simulink model "FAST_11TO14mpers"  (R2019a)
settings: Solver=FixedStepAuto  StartTime=0.0  StopTime=400  FixedStep=DT  RelTol=1e-3
values from neighbouring files (symbols this model uses):
  Control = struct    [testqLPV.m]
  Drivetrain = struct    [dataDLR.m]
  OutList = OutTable.Properties.VariableNames    [initLPVParam.m]    (also in testCtrl.m; testOutList.m = cell(40, 1); testqLPV.m = cell(40, 1))
undefined symbols (not defined in the file or in its folder): CertificationSettings, DiscIntNeverNeededParam, P_InitAngle, RPM_Init, strmatch
settings Model: ExtModeTrigMode=oneshot  ExtModeArmWhenConnect=off  Creator=Hazim Namik  LastModifiedBy=ditt_aj
settings DataIOCC: LimitDataPoints=on  SaveFormat=Array  ReturnWorkspaceOutputs=off
settings OptimizationCC: BlockReduction=off  BooleanDataType=off  LifeSpan=inf
settings DebuggingCC: SaveWithParameterizedLinksMsg=none  UnderspecifiedInitializationDetection=Classic  MergeDetectMultiDrivingBlocksExec=none  SignalResolutionControl=TryResolveAllWithWarning  SFUnexpectedBacktrackingDiag=warning  SFNoUnconditionalDefaultTransitionDiag=warning  SFExecutionAtInitializationDiag=none  ArithmeticOperatorsInVariantConditions=warning
settings HardwareCC: ProdBitPerPointer=32  ProdBitPerSizeT=32  ProdBitPerPtrDiffT=32  ProdLargestAtomicFloat=None  ProdIntDivRoundTo=Undefined  ProdEndianess=Unspecified  ProdWordSize=32  ProdHWDeviceType=32-bit Generic  TargetUnknown=on
settings ModelReferenceCC: PropagateSignalLabelsOutOfModel=off
settings SFSimCC: SimUseLocalCustomCode=off
settings RTWCC: RTWUseLocalCustomCode=off
settings CodeAppCC: StateflowObjectComments=on
settings GRTTargetCC: TargetLangStandard=C89/C90 (ANSI)  GeneratePreprocessorConditionals=Disable all
settings ConfigComp: CovMetricSettings=dw  CovHtmlReporting=on  CovSaveCumulativeToWorkspaceVar=on  CovSaveSingleToWorkspaceVar=on  CovExternalEMLEnable=off

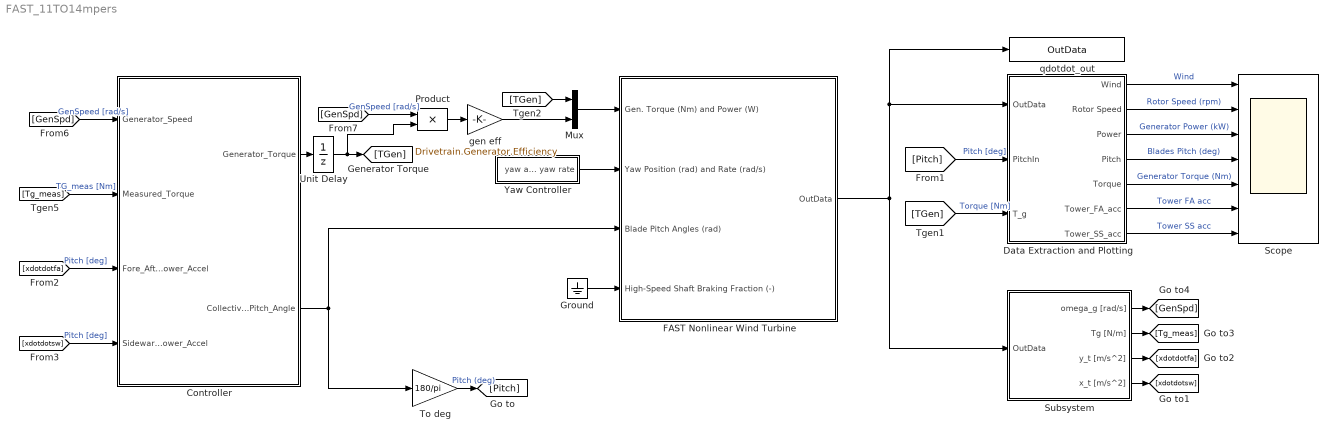
== system FAST_11TO14mpers ==
  Controller : Subsystem
  Data Extraction and Plotting : Subsystem
  FAST Nonlinear Wind Turbine : Subsystem  mask(FAST Nonlinear Wind Turbine){}
      mask help: This block contains the FAST S-Function.
      mask init:
      | clear FAST_SFunc
  Ground : Ground
  Mux : Mux  Inputs=2
  Product : Product  RndMeth=Zero
  Scope : Scope  NumInputPorts=7
      settings: Tag=Scope
  Subsystem : Subsystem
  To deg : Gain  Gain=180/pi
  Unit Delay : UnitDelay  InitialCondition=RPM_Init*Drivetrain.Gearbox.Ratio  SampleTime=-1  HasFrameUpgradeWarning=on
  Yaw Controller : Subsystem
  gen eff : Gain  Gain=Drivetrain.Generator.Efficiency
  qdotdot_out : ToWorkspace  VariableName=OutData  SampleTime=-1
  wires:
  Mux/1 -> FAST Nonlinear Wind Turbine/1(Gen. Torque (Nm) and Power (W))
  Yaw Controller/1(yaw and yaw rate) -> FAST Nonlinear Wind Turbine/2(Yaw Position (rad) and Rate (rad/s))
  To deg/1 -> [Pitch]  "Pitch (deg)"
  gen eff/1 -> Mux/2
  Product/1 -> gen eff/1
  Data Extraction and Plotting/3(Power) -> Scope/3  "Generator Power (kW)"
  [Pitch] -> Data Extraction and Plotting/2(PitchIn)  "Pitch [deg]"
  Data Extraction and Plotting/1(Wind) -> Scope/1  "Wind"
  Data Extraction and Plotting/2(Rotor Speed) -> Scope/2  "Rotor Speed (rpm)"
  [TGen] -> Data Extraction and Plotting/3(T_g)  "Torque [Nm]"
  FAST Nonlinear Wind Turbine/1(OutData) -> qdotdot_out/1, Data Extraction and Plotting/1(OutData), Subsystem/1(OutData)
  Data Extraction and Plotting/4(Pitch) -> Scope/4  "Blades Pitch (deg)"
  Data Extraction and Plotting/5(Torque) -> Scope/5  "Generator Torque (Nm)"
  Controller/1(Generator_Torque) -> Unit Delay/1
  Controller/2(Collective_Pitch_Angle) -> FAST Nonlinear Wind Turbine/3(Blade Pitch Angles (rad)), To deg/1
  Data Extraction and Plotting/6(Tower_FA_acc) -> Scope/6  "Tower FA acc"
  Data Extraction and Plotting/7(Tower_SS_acc) -> Scope/7  "Tower SS acc"
  Ground/1 -> FAST Nonlinear Wind Turbine/4(High-Speed Shaft Braking Fraction (-))
  [TGen] -> Mux/1
  Unit Delay/1 -> Product/2, [TGen]
  Subsystem/1(omega_g [rad/s]) -> [GenSpd]
  Subsystem/3(y_t [m/s^2]) -> [xdotdotfa]
  Subsystem/4(x_t [m/s^2]) -> [xdotdotsw]
  [GenSpd] -> Controller/1(Generator_Speed)  "GenSpeed [rad/s]"
  [Tg_meas] -> Controller/2(Measured_Torque)  "TG_meas [Nm]"
  [xdotdotsw] -> Controller/4(Sidewards_Tower_Accel)  "Pitch [deg]"
  [xdotdotfa] -> Controller/3(Fore_Aft_Tower_Accel)  "Pitch [deg]"
  Subsystem/2(Tg [N/m]) -> [Tg_meas]
  [GenSpd] -> Product/1  "GenSpeed [rad/s]"

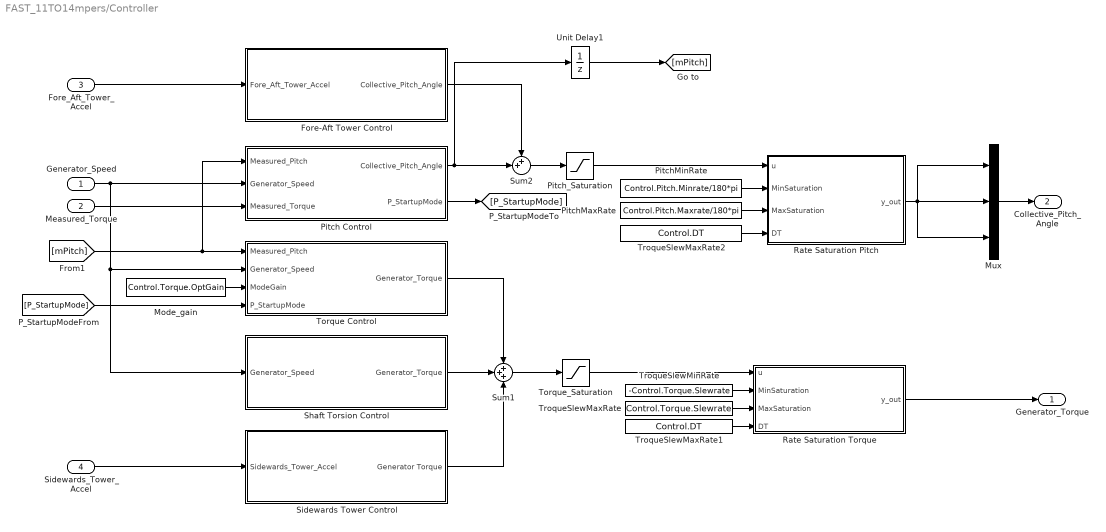
== system FAST_11TO14mpers/Controller ==
  Generator_Speed : Inport
  Measured_Torque : Inport  Port=2
  Fore_Aft_Tower_Accel : Inport  Port=3
  Sidewards_Tower_Accel : Inport  Port=4  PortDimensions=1
  Fore-Aft Tower Control : Subsystem
  Mode_gain : Constant  Value=Control.Torque.OptGain
  Mux : Mux  Inputs=3
  Pitch Control : Subsystem
  PitchMaxRate : Constant  Value=Control.Pitch.Maxrate/180*pi
  PitchMinRate : Constant  Value=Control.Pitch.Minrate/180*pi
  Pitch_Saturation : Saturate  UpperLimit=Control.Pitch.Max*pi/180  LowerLimit=Control.Pitch.Min*pi/180
  Rate Saturation Pitch : MATLAB Function  TreatAsAtomicUnit=on
  Rate Saturation Torque : MATLAB Function  TreatAsAtomicUnit=on
  Shaft Torsion Control : Subsystem
  Sidewards Tower Control : Subsystem
  Sum1 : Sum  Inputs=+++
  Sum2 : Sum  Inputs=++|
  Torque Control : Subsystem
  Torque_Saturation : Saturate  UpperLimit=Control.Torque.Limit  LowerLimit=Control.Torque.Min
  TroqueSlewMaxRate : Constant  Value=Control.Torque.Slewrate
  TroqueSlewMaxRate1 : Constant  Value=Control.DT
  TroqueSlewMaxRate2 : Constant  Value=Control.DT
  TroqueSlewMinRate : Constant  Value=-Control.Torque.Slewrate
  Unit Delay1 : UnitDelay  InitialCondition=P_InitAngle*pi/180  SampleTime=-1  HasFrameUpgradeWarning=on
  Generator_Torque : Outport
  Collective_Pitch_Angle : Outport  Port=2  PortDimensions=3
  wires:
  Sidewards_Tower_Accel/1 -> Sidewards Tower Control/1(Sidewards_Tower_Accel)
  Fore_Aft_Tower_Accel/1 -> Fore-Aft Tower Control/1(Fore_Aft_Tower_Accel)
  Fore-Aft Tower Control/1(Collective_Pitch_Angle) -> Sum2/1
  Torque Control/1(Generator_Torque) -> Sum1/1
  Sidewards Tower Control/1(Generator Torque) -> Sum1/3
  [mPitch] -> Pitch Control/1(Measured_Pitch), Torque Control/1(Measured_Pitch)
  Measured_Torque/1 -> Pitch Control/3(Measured_Torque)
  Shaft Torsion Control/1(Generator_Torque) -> Sum1/2
  Mode_gain/1 -> Torque Control/3(ModeGain)
  Sum1/1 -> Torque_Saturation/1
  Mux/1 -> Collective_Pitch_Angle/1
  Unit Delay1/1 -> [mPitch]
  Sum2/1 -> Pitch_Saturation/1
  Rate Saturation Pitch/1(y_out) -> Mux/3, Mux/2, Mux/1
  PitchMinRate/1 -> Rate Saturation Pitch/2(MinSaturation)
  PitchMaxRate/1 -> Rate Saturation Pitch/3(MaxSaturation)
  Pitch_Saturation/1 -> Rate Saturation Pitch/1(u)
  Torque_Saturation/1 -> Rate Saturation Torque/1(u)
  TroqueSlewMinRate/1 -> Rate Saturation Torque/2(MinSaturation)
  TroqueSlewMaxRate/1 -> Rate Saturation Torque/3(MaxSaturation)
  Generator_Speed/1 -> Pitch Control/2(Generator_Speed), Torque Control/2(Generator_Speed), Shaft Torsion Control/1(Generator_Speed)
  [P_StartupMode] -> Torque Control/4(P_StartupMode)
  Pitch Control/2(P_StartupMode) -> [P_StartupMode]
  Pitch Control/1(Collective_Pitch_Angle) -> Sum2/2, Unit Delay1/1
  Rate Saturation Torque/1(y_out) -> Generator_Torque/1
  TroqueSlewMaxRate1/1 -> Rate Saturation Torque/4(DT)
  TroqueSlewMaxRate2/1 -> Rate Saturation Pitch/4(DT)

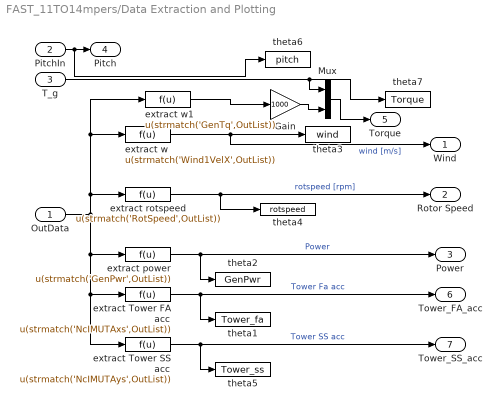
== system FAST_11TO14mpers/Data Extraction and Plotting ==
  OutData : Inport
  PitchIn : Inport  Port=2
  T_g : Inport  Port=3
  Gain : Gain  Gain=1000
  Mux : Mux  Inputs=2
  extract Tower FA acc : Fcn  Expr=u(strmatch('NcIMUTAxs',OutList))
  extract Tower SS acc : Fcn  Expr=u(strmatch('NcIMUTAys',OutList))
  extract power : Fcn  Expr=u(strmatch('GenPwr',OutList))
  extract rotspeed : Fcn  Expr=u(strmatch('RotSpeed',OutList))
  extract w : Fcn  Expr=u(strmatch('Wind1VelX',OutList))
  extract w1 : Fcn  Expr=u(strmatch('GenTq',OutList))
  theta1 : ToWorkspace  VariableName=Tower_fa  SampleTime=-1
      settings: MaxDataPoints=Inf  Decimation=3
  theta2 : ToWorkspace  VariableName=GenPwr  SampleTime=-1
      settings: MaxDataPoints=Inf  Decimation=3
  theta3 : ToWorkspace  VariableName=wind  SampleTime=-1
      settings: MaxDataPoints=Inf  Decimation=3
  theta4 : ToWorkspace  VariableName=rotspeed  SampleTime=-1
      settings: MaxDataPoints=Inf  Decimation=3
  theta5 : ToWorkspace  VariableName=Tower_ss  SampleTime=-1
      settings: MaxDataPoints=Inf  Decimation=3
  theta6 : ToWorkspace  VariableName=pitch  SampleTime=-1
      settings: MaxDataPoints=Inf  Decimation=3
  theta7 : ToWorkspace  VariableName=Torque  SampleTime=-1
      settings: MaxDataPoints=Inf  Decimation=3
  Wind : Outport
  Rotor Speed : Outport  Port=2
  Power : Outport  Port=3
  Pitch : Outport  Port=4
  Torque : Outport  Port=5
  Tower_FA_acc : Outport  Port=6
  Tower_SS_acc : Outport  Port=7
  wires:
  extract w/1 -> Wind/1, theta3/1  "wind [m/s]"
  extract rotspeed/1 -> theta4/1, Rotor Speed/1  "rotspeed [rpm]"
  extract power/1 -> theta2/1, Power/1  "Power"
  PitchIn/1 -> theta6/1, Pitch/1
  T_g/1 -> Mux/1, theta7/1
  extract Tower FA acc/1 -> theta1/1, Tower_FA_acc/1  "Tower Fa acc"
  OutData/1 -> extract w/1, extract w1/1, extract rotspeed/1, extract Tower SS acc/1, extract Tower FA acc/1, extract power/1
  extract Tower SS acc/1 -> theta5/1, Tower_SS_acc/1  "Tower SS acc"
  extract w1/1 -> Gain/1
  Gain/1 -> Mux/2
  Mux/1 -> Torque/1

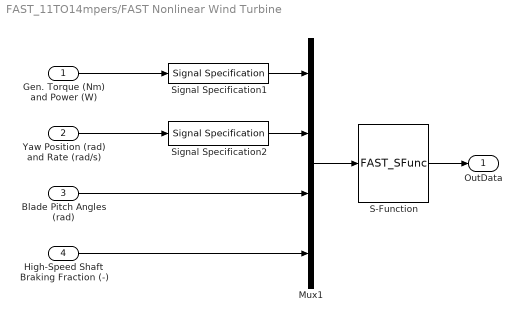
== system FAST_11TO14mpers/FAST Nonlinear Wind Turbine ==
  Gen. Torque (Nm) and Power (W) : Inport
  Yaw Position (rad) and Rate (rad/s) : Inport  Port=2
  Blade Pitch Angles (rad) : Inport  Port=3
  High-Speed Shaft Braking Fraction (-) : Inport  Port=4
  Mux1 : Mux
  S-Function : S-Function  FunctionName=FAST_SFunc  Parameters=FAST_InputFileName, TMax, 0  SFunctionDeploymentMode=off  EnableBusSupport=off
  Signal Specification1 : SignalSpecification  OutDataTypeStr=double  Dimensions=2
  Signal Specification2 : SignalSpecification  OutDataTypeStr=double  Dimensions=2
  OutData : Outport
  wires:
  Gen. Torque (Nm) and Power (W)/1 -> Signal Specification1/1
  S-Function/1 -> OutData/1
  Mux1/1 -> S-Function/1
  Blade Pitch Angles (rad)/1 -> Mux1/3
  Yaw Position (rad) and Rate (rad/s)/1 -> Signal Specification2/1
  Signal Specification1/1 -> Mux1/1
  Signal Specification2/1 -> Mux1/2
  High-Speed Shaft Braking Fraction (-)/1 -> Mux1/4

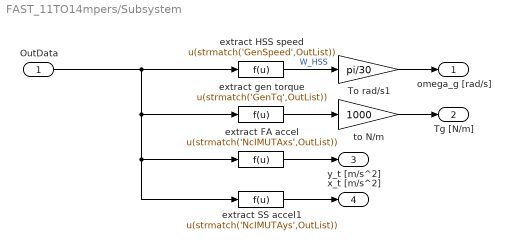
== system FAST_11TO14mpers/Subsystem ==
  OutData : Inport
  To rad/s1 : Gain  Gain=pi/30
  extract FA accel : Fcn  Expr=u(strmatch('NcIMUTAxs',OutList))
  extract HSS speed : Fcn  Expr=u(strmatch('GenSpeed',OutList))
  extract SS accel1 : Fcn  Expr=u(strmatch('NcIMUTAys',OutList))
  extract gen torque : Fcn  Expr=u(strmatch('GenTq',OutList))
  to N/m : Gain  Gain=1000
  omega_g [rad/s] : Outport
  Tg [N/m] : Outport  Port=2
  y_t [m/s^2] : Outport  Port=3
  x_t [m/s^2] : Outport  Port=4
  wires:
  to N/m/1 -> Tg [N/m]/1
  OutData/1 -> extract SS accel1/1, extract FA accel/1, extract gen torque/1, extract HSS speed/1
  extract FA accel/1 -> y_t [m/s^2]/1
  extract HSS speed/1 -> To rad/s1/1  "W_HSS"
  extract gen torque/1 -> to N/m/1
  extract SS accel1/1 -> x_t [m/s^2]/1
  To rad/s1/1 -> omega_g [rad/s]/1

== system FAST_11TO14mpers/Yaw Controller ==
  Mux : Mux  Inputs=2
  Yaw Position : Constant  Value=0
  Yaw rate : Constant  Value=0
  yaw and yaw rate : Outport
  wires:
  Mux/1 -> yaw and yaw rate/1
  Yaw Position/1 -> Mux/1
  Yaw rate/1 -> Mux/2

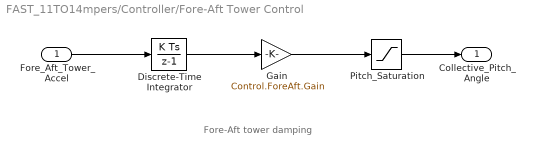
== system FAST_11TO14mpers/Controller/Fore-Aft Tower Control ==
  note: Fore-Aft tower damping
  Fore_Aft_Tower_Accel : Inport
  Discrete-Time Integrator : DiscreteIntegrator  SampleTime=-1  ICPrevOutput=DiscIntNeverNeededParam  ICPrevScaledInput=DiscIntNeverNeededParam
  Gain : Gain  Gain=Control.ForeAft.Gain
  Pitch_Saturation : Saturate  UpperLimit=Control.ForeAft.MaxPitchAmplitude*pi/180  LowerLimit=-Control.ForeAft.MaxPitchAmplitude*pi/180
  Collective_Pitch_Angle : Outport
  wires:
  Fore_Aft_Tower_Accel/1 -> Discrete-Time Integrator/1
  Pitch_Saturation/1 -> Collective_Pitch_Angle/1
  Discrete-Time Integrator/1 -> Gain/1
  Gain/1 -> Pitch_Saturation/1

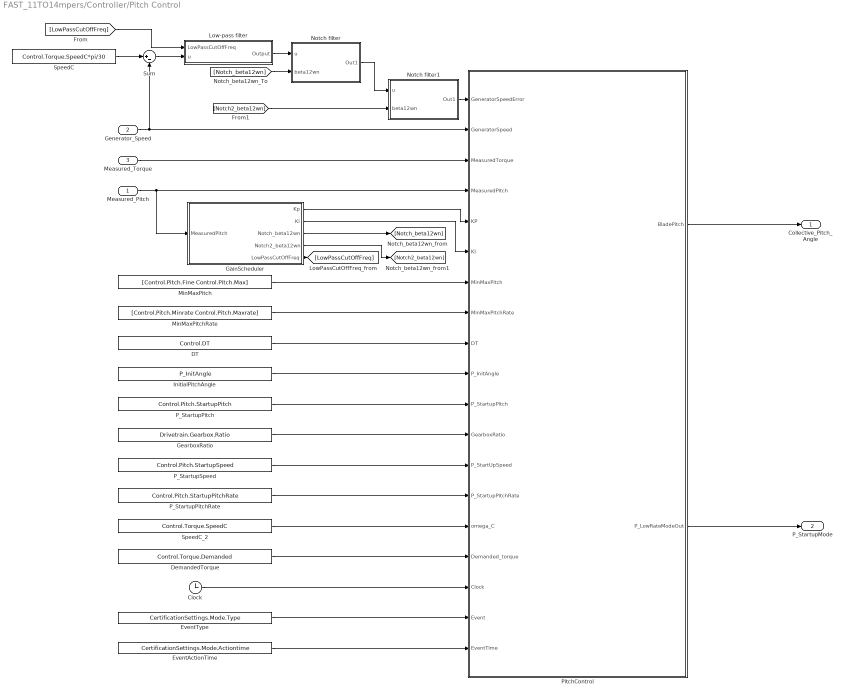
== system FAST_11TO14mpers/Controller/Pitch Control ==
  Measured_Pitch : Inport
  Generator_Speed : Inport  Port=2
  Measured_Torque : Inport  Port=3
  Clock : Clock
  DT : Constant  Value=Control.DT
  DemandedTorque : Constant  Value=Control.Torque.Demanded
  EventActionTime : Constant  Value=CertificationSettings.Mode.Actiontime
  EventType : Constant  Value=CertificationSettings.Mode.Type
  GainScheduler : Subsystem
  GearboxRatio : Constant  Value=Drivetrain.Gearbox.Ratio
  InitialPitchAngle : Constant  Value=P_InitAngle
  Low-pass filter : Subsystem
  MinMaxPitch : Constant  Value=[Control.Pitch.Fine Control.Pitch.Max]
  MinMaxPitchRate : Constant  Value=[Control.Pitch.Minrate Control.Pitch.Maxrate]
  Notch filter : Subsystem
  Notch filter1 : Subsystem
  P_StartupPitch : Constant  Value=Control.Pitch.StartupPitch
  P_StartupPitchRate : Constant  Value=Control.Pitch.StartupPitchRate
  P_StartupSpeed : Constant  Value=Control.Pitch.StartupSpeed
  PitchControl : MATLAB Function  TreatAsAtomicUnit=on
  SpeedC : Constant  Value=Control.Torque.SpeedC*pi/30
  SpeedC_2 : Constant  Value=Control.Torque.SpeedC
  Sum : Sum  Inputs=|+-
  Collective_Pitch_Angle : Outport
  P_StartupMode : Outport  Port=2
  wires:
  MinMaxPitch/1 -> PitchControl/7(MinMaxPitch)
  MinMaxPitchRate/1 -> PitchControl/8(MinMaxPitchRate)
  PitchControl/1(BladePitch) -> Collective_Pitch_Angle/1
  Measured_Torque/1 -> PitchControl/3(MeasuredTorque)
  SpeedC/1 -> Sum/1
  Generator_Speed/1 -> PitchControl/2(GeneratorSpeed), Sum/2
  Sum/1 -> Low-pass filter/2(u)
  PitchControl/2(P_LowRateModeOut) -> P_StartupMode/1
  DT/1 -> PitchControl/9(DT)
  P_StartupPitch/1 -> PitchControl/11(P_StartupPitch)
  InitialPitchAngle/1 -> PitchControl/10(P_InitAngle)
  GearboxRatio/1 -> PitchControl/12(GearboxRatio)
  P_StartupSpeed/1 -> PitchControl/13(P_StartUpSpeed)
  P_StartupPitchRate/1 -> PitchControl/14(P_StartupPitchRate)
  SpeedC_2/1 -> PitchControl/15(omega_C)
  DemandedTorque/1 -> PitchControl/16(Demanded_torque)
  Measured_Pitch/1 -> GainScheduler/1(MeasuredPitch), PitchControl/4(MeasuredPitch)
  EventType/1 -> PitchControl/18(Event)
  Clock/1 -> PitchControl/17(Clock)
  EventActionTime/1 -> PitchControl/19(EventTime)
  GainScheduler/1(Kp) -> PitchControl/5(KP)
  GainScheduler/2(Ki) -> PitchControl/6(KI)
  [Notch_beta12wn] -> Notch filter/2(beta12wn)
  GainScheduler/3(Notch_beta12wn) -> [Notch_beta12wn]
  Low-pass filter/1(Output) -> Notch filter/1(u)
  Notch filter/1(Out1) -> Notch filter1/1(u)
  GainScheduler/5(LowPassCutOffFreq) -> [LowPassCutOffFreq]
  [LowPassCutOffFreq] -> Low-pass filter/1(LowPassCutOffFreq)
  GainScheduler/4(Notch2_beta12wn) -> [Notch2_beta12wn]
  [Notch2_beta12wn] -> Notch filter1/2(beta12wn)
  Notch filter1/1(Out1) -> PitchControl/1(GeneratorSpeedError)

== system FAST_11TO14mpers/Controller/Shaft Torsion Control ==
  Generator_Speed : Inport
  Gain : Gain  Gain=0
  Generator_Torque : Outport
  wires:
  Generator_Speed/1 -> Gain/1
  Gain/1 -> Generator_Torque/1

== system FAST_11TO14mpers/Controller/Sidewards Tower Control ==
  Sidewards_Tower_Accel : Inport
  Gain : Gain  Gain=0
  Generator Torque : Outport
  wires:
  Sidewards_Tower_Accel/1 -> Gain/1
  Gain/1 -> Generator Torque/1

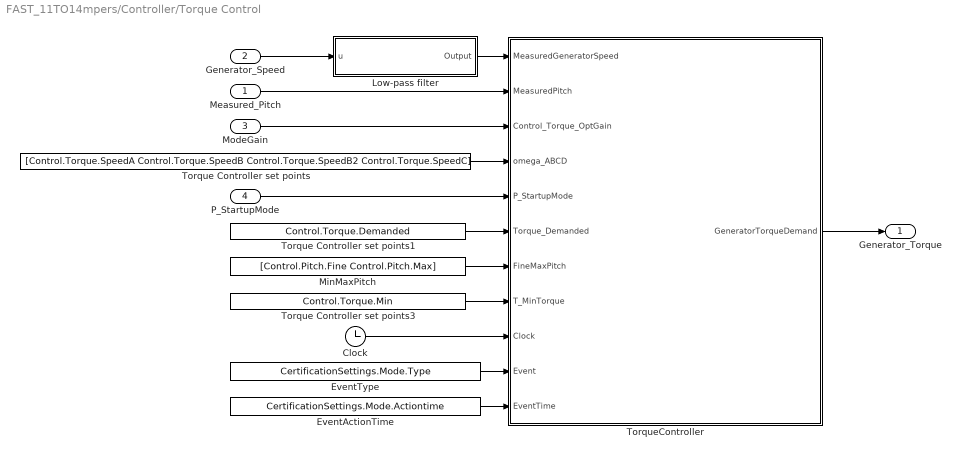
== system FAST_11TO14mpers/Controller/Torque Control ==
  Measured_Pitch : Inport
  Generator_Speed : Inport  Port=2
  ModeGain : Inport  Port=3
  P_StartupMode : Inport  Port=4
  Clock : Clock
  EventActionTime : Constant  Value=CertificationSettings.Mode.Actiontime
  EventType : Constant  Value=CertificationSettings.Mode.Type
  Low-pass filter : Subsystem
  MinMaxPitch : Constant  Value=[Control.Pitch.Fine Control.Pitch.Max]
  Torque Controller set points : Constant  Value=[Control.Torque.SpeedA Control.Torque.SpeedB Control.Torque.SpeedB2 Control.Torque.SpeedC]
  Torque Controller set points1 : Constant  Value=Control.Torque.Demanded
  Torque Controller set points3 : Constant  Value=Control.Torque.Min
  TorqueController : MATLAB Function  TreatAsAtomicUnit=on
  Generator_Torque : Outport
  wires:
  Generator_Speed/1 -> Low-pass filter/1(u)
  TorqueController/1(GeneratorTorqueDemand) -> Generator_Torque/1
  Measured_Pitch/1 -> TorqueController/2(MeasuredPitch)
  ModeGain/1 -> TorqueController/3(Control_Torque_OptGain)
  Torque Controller set points/1 -> TorqueController/4(omega_ABCD)
  P_StartupMode/1 -> TorqueController/5(P_StartupMode)
  Low-pass filter/1(Output) -> TorqueController/1(MeasuredGeneratorSpeed)
  Torque Controller set points3/1 -> TorqueController/8(T_MinTorque)
  MinMaxPitch/1 -> TorqueController/7(FineMaxPitch)
  Torque Controller set points1/1 -> TorqueController/6(Torque_Demanded)
  Clock/1 -> TorqueController/9(Clock)
  EventType/1 -> TorqueController/10(Event)
  EventActionTime/1 -> TorqueController/11(EventTime)

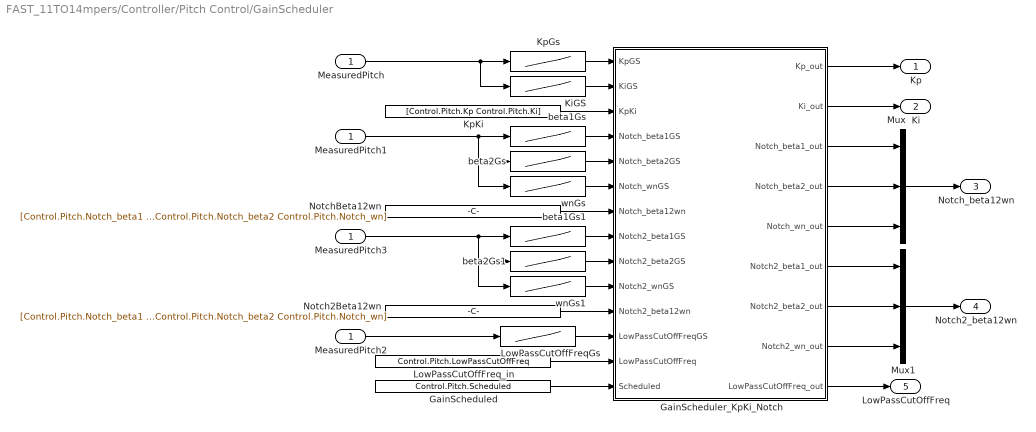
== system FAST_11TO14mpers/Controller/Pitch Control/GainScheduler ==
  MeasuredPitch : Inport
  GainScheduled : Constant  Value=Control.Pitch.Scheduled
  GainScheduler_KpKi_Notch : MATLAB Function  TreatAsAtomicUnit=on
  KiGS : Lookup_n-D  NumberOfTableDimensions=1  BreakpointsForDimension1=Control.Pitch.ScheduledPitchAngles  Table=Control.Pitch.KiGS  ExtrapMethod=Clip  UseLastTableValue=on  InternalRulePriority=Speed  RndMeth=Simplest  InputSameDT=on
  KpGs : Lookup_n-D  NumberOfTableDimensions=1  BreakpointsForDimension1=Control.Pitch.ScheduledPitchAngles  Table=Control.Pitch.KpGS  ExtrapMethod=Clip  UseLastTableValue=on  InternalRulePriority=Speed  RndMeth=Simplest  InputSameDT=on
  KpKi : Constant  Value=[Control.Pitch.Kp Control.Pitch.Ki]
  LowPassCutOffFreqGs : Lookup_n-D  NumberOfTableDimensions=1  BreakpointsForDimension1=Control.Pitch.ScheduledPitchAngles  Table=Control.Pitch.LowPassCutOffFreqGS  ExtrapMethod=Clip  UseLastTableValue=on  InternalRulePriority=Speed  RndMeth=Simplest  InputSameDT=on
  LowPassCutOffFreq_in : Constant  Value=Control.Pitch.LowPassCutOffFreq
  MeasuredPitch1 : InportShadow
  MeasuredPitch2 : InportShadow
  MeasuredPitch3 : InportShadow
  Mux : Mux  Inputs=3
  Mux1 : Mux  Inputs=3
  Notch2Beta12wn : Constant  Value=[Control.Pitch.Notch_beta1 Control.Pitch.Notch_beta2 Control.Pitch.Notch_wn]
  NotchBeta12wn : Constant  Value=[Control.Pitch.Notch_beta1 Control.Pitch.Notch_beta2 Control.Pitch.Notch_wn]
  beta1Gs : Lookup_n-D  NumberOfTableDimensions=1  BreakpointsForDimension1=Control.Pitch.ScheduledPitchAngles  Table=Control.Pitch.Notch_beta1GS  ExtrapMethod=Clip  UseLastTableValue=on  InternalRulePriority=Speed  RndMeth=Simplest  InputSameDT=on
  beta1Gs1 : Lookup_n-D  NumberOfTableDimensions=1  BreakpointsForDimension1=Control.Pitch.ScheduledPitchAngles  Table=Control.Pitch.Notch2_beta1GS  ExtrapMethod=Clip  UseLastTableValue=on  InternalRulePriority=Speed  RndMeth=Simplest  InputSameDT=on
  beta2Gs : Lookup_n-D  NumberOfTableDimensions=1  BreakpointsForDimension1=Control.Pitch.ScheduledPitchAngles  Table=Control.Pitch.Notch_beta2GS  ExtrapMethod=Clip  UseLastTableValue=on  InternalRulePriority=Speed  RndMeth=Simplest  InputSameDT=on
  beta2Gs1 : Lookup_n-D  NumberOfTableDimensions=1  BreakpointsForDimension1=Control.Pitch.ScheduledPitchAngles  Table=Control.Pitch.Notch2_beta2GS  ExtrapMethod=Clip  UseLastTableValue=on  InternalRulePriority=Speed  RndMeth=Simplest  InputSameDT=on
  wnGs : Lookup_n-D  NumberOfTableDimensions=1  BreakpointsForDimension1=Control.Pitch.ScheduledPitchAngles  Table=Control.Pitch.Notch_wnGS  ExtrapMethod=Clip  UseLastTableValue=on  InternalRulePriority=Speed  RndMeth=Simplest  InputSameDT=on
  wnGs1 : Lookup_n-D  NumberOfTableDimensions=1  BreakpointsForDimension1=Control.Pitch.ScheduledPitchAngles  Table=Control.Pitch.Notch2_wnGS  ExtrapMethod=Clip  UseLastTableValue=on  InternalRulePriority=Speed  RndMeth=Simplest  InputSameDT=on
  Kp : Outport
  Ki : Outport  Port=2
  Notch_beta12wn : Outport  Port=3
  Notch2_beta12wn : Outport  Port=4
  LowPassCutOffFreq : Outport  Port=5
  wires:
  MeasuredPitch/1 -> KiGS/1, KpGs/1
  GainScheduled/1 -> GainScheduler_KpKi_Notch/14(Scheduled)
  GainScheduler_KpKi_Notch/2(Ki_out) -> Ki/1
  KpKi/1 -> GainScheduler_KpKi_Notch/3(KpKi)
  KpGs/1 -> GainScheduler_KpKi_Notch/1(KpGS)
  KiGS/1 -> GainScheduler_KpKi_Notch/2(KiGS)
  GainScheduler_KpKi_Notch/1(Kp_out) -> Kp/1
  GainScheduler_KpKi_Notch/3(Notch_beta1_out) -> Mux/1
  GainScheduler_KpKi_Notch/4(Notch_beta2_out) -> Mux/2
  GainScheduler_KpKi_Notch/5(Notch_wn_out) -> Mux/3
  NotchBeta12wn/1 -> GainScheduler_KpKi_Notch/7(Notch_beta12wn)
  MeasuredPitch1/1 -> wnGs/1, beta2Gs/1, beta1Gs/1
  beta1Gs/1 -> GainScheduler_KpKi_Notch/4(Notch_beta1GS)
  beta2Gs/1 -> GainScheduler_KpKi_Notch/5(Notch_beta2GS)
  wnGs/1 -> GainScheduler_KpKi_Notch/6(Notch_wnGS)
  Mux/1 -> Notch_beta12wn/1
  MeasuredPitch2/1 -> LowPassCutOffFreqGs/1
  LowPassCutOffFreqGs/1 -> GainScheduler_KpKi_Notch/12(LowPassCutOffFreqGS)
  LowPassCutOffFreq_in/1 -> GainScheduler_KpKi_Notch/13(LowPassCutOffFreq)
  GainScheduler_KpKi_Notch/9(LowPassCutOffFreq_out) -> LowPassCutOffFreq/1
  GainScheduler_KpKi_Notch/7(Notch2_beta2_out) -> Mux1/2
  Mux1/1 -> Notch2_beta12wn/1
  GainScheduler_KpKi_Notch/6(Notch2_beta1_out) -> Mux1/1
  GainScheduler_KpKi_Notch/8(Notch2_wn_out) -> Mux1/3
  MeasuredPitch3/1 -> wnGs1/1, beta2Gs1/1, beta1Gs1/1
  beta1Gs1/1 -> GainScheduler_KpKi_Notch/8(Notch2_beta1GS)
  beta2Gs1/1 -> GainScheduler_KpKi_Notch/9(Notch2_beta2GS)
  wnGs1/1 -> GainScheduler_KpKi_Notch/10(Notch2_wnGS)
  Notch2Beta12wn/1 -> GainScheduler_KpKi_Notch/11(Notch2_beta12wn)

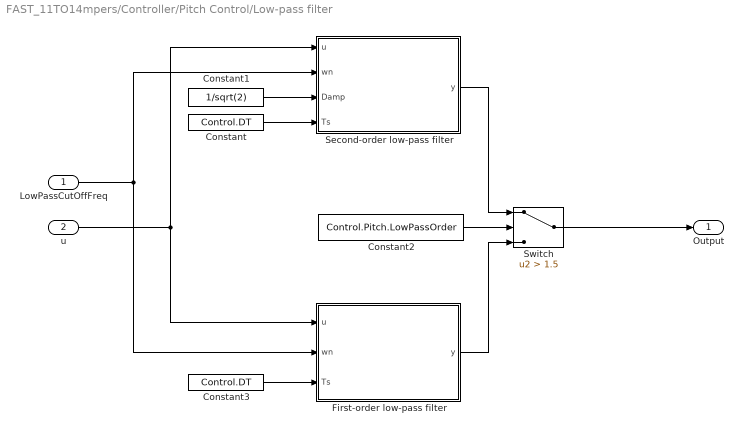
== system FAST_11TO14mpers/Controller/Pitch Control/Low-pass filter ==
  LowPassCutOffFreq : Inport
  u : Inport  Port=2
  Constant : Constant  Value=Control.DT
  Constant1 : Constant  Value=1/sqrt(2)
  Constant2 : Constant  Value=Control.Pitch.LowPassOrder
  Constant3 : Constant  Value=Control.DT
  First-order low-pass filter : MATLAB Function  TreatAsAtomicUnit=on
  Second-order low-pass filter : MATLAB Function  TreatAsAtomicUnit=on
  Switch : Switch  Criteria=u2 > Threshold  Threshold=1.5
  Output : Outport
  wires:
  Switch/1 -> Output/1
  Constant1/1 -> Second-order low-pass filter/3(Damp)
  Constant/1 -> Second-order low-pass filter/4(Ts)
  Constant3/1 -> First-order low-pass filter/3(Ts)
  Constant2/1 -> Switch/2
  First-order low-pass filter/1(y) -> Switch/3
  Second-order low-pass filter/1(y) -> Switch/1
  LowPassCutOffFreq/1 -> Second-order low-pass filter/2(wn), First-order low-pass filter/2(wn)
  u/1 -> First-order low-pass filter/1(u), Second-order low-pass filter/1(u)

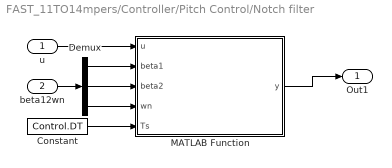
== system FAST_11TO14mpers/Controller/Pitch Control/Notch filter ==
  u : Inport
  beta12wn : Inport  Port=2
  Constant : Constant  Value=Control.DT
  Demux : Demux  Outputs=3
  MATLAB Function : MATLAB Function  TreatAsAtomicUnit=on
  Out1 : Outport
  wires:
  MATLAB Function/1(y) -> Out1/1
  Demux/1 -> MATLAB Function/2(beta1)
  Demux/2 -> MATLAB Function/3(beta2)
  Demux/3 -> MATLAB Function/4(wn)
  beta12wn/1 -> Demux/1
  u/1 -> MATLAB Function/1(u)
  Constant/1 -> MATLAB Function/5(Ts)

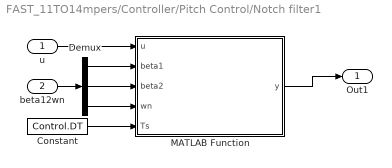
== system FAST_11TO14mpers/Controller/Pitch Control/Notch filter1 ==
  u : Inport
  beta12wn : Inport  Port=2
  Constant : Constant  Value=Control.DT
  Demux : Demux  Outputs=3
  MATLAB Function : MATLAB Function  TreatAsAtomicUnit=on
  Out1 : Outport
  wires:
  MATLAB Function/1(y) -> Out1/1
  Demux/1 -> MATLAB Function/2(beta1)
  Demux/2 -> MATLAB Function/3(beta2)
  Demux/3 -> MATLAB Function/4(wn)
  beta12wn/1 -> Demux/1
  u/1 -> MATLAB Function/1(u)
  Constant/1 -> MATLAB Function/5(Ts)

== system FAST_11TO14mpers/Controller/Torque Control/Low-pass filter ==
  u : Inport
  Constant1 : Constant  Value=Control.Torque.LowPassCutOffFreq
  Constant3 : Constant  Value=Control.DT
  First-order low-pass filter : MATLAB Function  TreatAsAtomicUnit=on
  Output : Outport
  wires:
  Constant3/1 -> First-order low-pass filter/3(Ts)
  u/1 -> First-order low-pass filter/1(u)
  First-order low-pass filter/1(y) -> Output/1
  Constant1/1 -> First-order low-pass filter/2(wn)

== matlab function FAST_11TO14mpers/Controller/Rate Saturation Torque ==
  data: u input; MinSaturation input; y_out output; MaxSaturation input; DT input
function y_out = fcn(u, MinSaturation, MaxSaturation, DT)
persistent y

if isempty(y)
    y = u;
end

rate = (u-y)/DT;
rate = min(max(rate, MinSaturation), MaxSaturation);

y = y + rate*DT;
y_out = y;

== matlab function FAST_11TO14mpers/Controller/Rate Saturation Pitch ==
  data: u input; MinSaturation input; y_out output; MaxSaturation input; DT input
function y_out = fcn(u, MinSaturation, MaxSaturation, DT)
persistent y

if isempty(y)
    y = u;
end

rate = (u-y)/DT;
rate = min(max(rate, MinSaturation), MaxSaturation);

y = y + rate*DT;
y_out = y;

== matlab function FAST_11TO14mpers/Controller/Torque Control/TorqueController ==
  data: GeneratorTorqueDemand output; MeasuredGeneratorSpeed input; MeasuredPitch input; Control_Torque_OptGain input; omega_ABCD input size=[1 4]; P_StartupMode input; Torque_Demanded input; FineMaxPitch input; T_MinTorque input; Clock input; Event input; EventTime input
function GeneratorTorqueDemand  = TorqueController(MeasuredGeneratorSpeed, MeasuredPitch, Control_Torque_OptGain, omega_ABCD, P_StartupMode, Torque_Demanded, FineMaxPitch, T_MinTorque, Clock, Event, EventTime)

% Calculate generator torque setpoint according to the feedforward wind
% turbine control law T = K*\omega^2
GeneratorTorqueDemand = max(min(Control_Torque_OptGain*MeasuredGeneratorSpeed^2, Torque_Demanded), T_MinTorque);

% Calculate torques at beginning and end of CP_max operation
TorqueOmegaB = Control_Torque_OptGain*(omega_ABCD(2)*pi/30)^2;
TorqueOmegaC = Control_Torque_OptGain*(omega_ABCD(3)*pi/30)^2;

% Apply maximum demanded torque when pitch is 1 degree above fine-pitch and
% the wind turbine is not in start-up mode.
if (Event == 5 && Clock >= EventTime) && (MeasuredPitch > (FineMaxPitch(2) - 1.0)*pi/180) %Emergency shutdown
    GeneratorTorqueDemand = 0.0;
elseif MeasuredPitch > (FineMaxPitch(1) + 1.0)*pi/180 && P_StartupMode == false
    GeneratorTorqueDemand = Torque_Demanded;
elseif MeasuredGeneratorSpeed < omega_ABCD(1)*pi/30
    GeneratorTorqueDemand = T_MinTorque;
elseif MeasuredGeneratorSpeed < omega_ABCD(2)*pi/30
    GeneratorTorqueDemand = (TorqueOmegaB - T_MinTorque)/((omega_ABCD(2) - omega_ABCD(1))*pi/30)*(MeasuredGeneratorSpeed - omega_ABCD(1)*pi/30) + T_MinTorque;
elseif MeasuredGeneratorSpeed >= omega_ABCD(3)*pi/30
    GeneratorTorqueDemand = (Torque_Demanded - TorqueOmegaC)/((omega_ABCD(4) - omega_ABCD(3))*pi/30)*(MeasuredGeneratorSpeed - omega_ABCD(3)*pi/30) + TorqueOmegaC;
end

== matlab function FAST_11TO14mpers/Controller/Pitch Control/PitchControl ==
  settings: updateMethod=DISCRETE  sampleTime=Control.DT
  data: GeneratorSpeedError input; GeneratorSpeed input; MeasuredTorque input; MeasuredPitch input; BladePitch output; KP input; KI input; MinMaxPitch input; MinMaxPitchRate input; DT input; P_InitAngle input; P_StartupPitch input; GearboxRatio input; P_StartUpSpeed input; P_StartupPitchRate input; omega_C input; Demanded_torque input; Clock input; P_LowRateModeOut output boolean; Event input; EventTime input
function [BladePitch, P_LowRateModeOut]  = PitchControl(GeneratorSpeedError, GeneratorSpeed, MeasuredTorque, MeasuredPitch, KP, KI, MinMaxPitch, MinMaxPitchRate, DT, P_InitAngle, P_StartupPitch, GearboxRatio, P_StartUpSpeed, P_StartupPitchRate, omega_C, Demanded_torque, Clock, Event, EventTime)
persistent I_term PI_term_old P_LowRateMode P_LowRateMode_old

%Initialize all persistent variables
if isempty(I_term)
    I_term = (P_InitAngle*pi/180);
    PI_term_old = (P_InitAngle*pi/180);
    P_LowRateMode = true;
    P_LowRateMode_old = true; %Used to detect change from start-up/below-rated to above-rated operation mode
end

%Event handling part
if (Event == 2 && Clock >= EventTime) || (Event == 5 && Clock >= EventTime) %Grid loss, emergency shutdown
    P_LowRateMode = false;
    P_MinPitchSat = MinMaxPitch(2)*pi/180;
elseif (Event == 4 && Clock >= EventTime) % Normal shutdown
    P_LowRateMode = true;
    P_MinPitchSat = MinMaxPitch(2)*pi/180;
elseif Event == 7 || Event == 6 % Idling and parked mode
    P_MinPitchSat = MinMaxPitch(2)*pi/180;
elseif MeasuredTorque > Demanded_torque*0.99 || GeneratorSpeed > omega_C*(pi/30) % Above-rated operating mode
    P_LowRateMode = false;
    P_MinPitchSat = MinMaxPitch(1)*pi/180;
    if P_LowRateMode ~= P_LowRateMode_old % On switching event between below-rated to above rated, reinitialize the integral term to ensure smooth transition
        I_term = MeasuredPitch;
    end
elseif Event == 3 || GeneratorSpeed < P_StartUpSpeed*GearboxRatio*(pi/30) % Normal startup 
    if Event == 3 && Clock < EventTime
        P_LowRateMode = true;
        P_MinPitchSat = MinMaxPitch(2)*pi/180;
    elseif (Event == 3 && Clock >= EventTime) && (GeneratorSpeed < P_StartUpSpeed*GearboxRatio*(pi/30))
        P_LowRateMode = true;
        P_MinPitchSat = P_StartupPitch*pi/180;
    else
        P_LowRateMode = true;
        P_MinPitchSat = MinMaxPitch(1)*pi/180;
    end
else
    P_MinPitchSat = MinMaxPitch(1)*pi/180;
end
 
% Pitch controller, KP and KI are constant or gain-scheduled, depending on
% input. Integral term is saturated, lower bound is variable and depends on
% event or operatinig mode.
P_term = KP*GeneratorSpeedError;
I_term = I_term + KI*GeneratorSpeedError*DT;
I_term = min(max(I_term,P_MinPitchSat), MinMaxPitch(2)*pi/180);

PI_term = P_term + I_term;
PI_term_sat = min(max(PI_term,P_MinPitchSat), MinMaxPitch(2)*pi/180);

% Calculate and limit pitch rate. Limit on rate is subject to event or
% operating mode.
PitchRate = (PI_term_sat - PI_term_old)/DT;
if P_LowRateMode
    PitchRate = min(max(PitchRate, -P_StartupPitchRate*pi/180), P_StartupPitchRate*pi/180);
else
    PitchRate = min(max(PitchRate, MinMaxPitchRate(1)*pi/180), MinMaxPitchRate(2)*pi/180);
end
BladePitch = PI_term_old + PitchRate*DT;

% Write variables to persistent variables and/or outputs
PI_term_old = BladePitch;
P_LowRateModeOut = P_LowRateMode;
P_LowRateMode_old = P_LowRateMode;
end

== matlab function FAST_11TO14mpers/Controller/Pitch Control/GainScheduler/GainScheduler_KpKi_Notch ==
  data: KpGS input; KiGS input; Kp_out output; KpKi input; Notch_beta1GS input; Notch_beta2GS input; Notch_wnGS input; Notch_beta12wn input; Notch2_beta1GS input; Notch2_beta2GS input; Notch2_wnGS input; Notch2_beta12wn input; LowPassCutOffFreqGS input; LowPassCutOffFreq input; Scheduled input; Ki_out output; Notch_beta1_out output; Notch_beta2_out output; Notch_wn_out output; Notch2_beta1_out output; Notch2_beta2_out output; Notch2_wn_out output; LowPassCutOffFreq_out output
function [Kp_out, Ki_out, Notch_beta1_out, Notch_beta2_out, Notch_wn_out, Notch2_beta1_out, Notch2_beta2_out, Notch2_wn_out, LowPassCutOffFreq_out] = fcn(KpGS, KiGS, KpKi, Notch_beta1GS, Notch_beta2GS, Notch_wnGS, Notch_beta12wn, Notch2_beta1GS, Notch2_beta2GS, Notch2_wnGS, Notch2_beta12wn, LowPassCutOffFreqGS, LowPassCutOffFreq, Scheduled)

if Scheduled > 0.5
    Kp_out = KpGS;
    Ki_out = KiGS;
    Notch_beta1_out = Notch_beta1GS;
    Notch_beta2_out = Notch_beta2GS;
    Notch_wn_out = Notch_wnGS;
    Notch2_beta1_out = Notch2_beta1GS;
    Notch2_beta2_out = Notch2_beta2GS;
    Notch2_wn_out = Notch2_wnGS;
    LowPassCutOffFreq_out = LowPassCutOffFreqGS;
else
    Kp_out = KpKi(1);
    Ki_out = KpKi(2);
    Notch_beta1_out = Notch_beta12wn(1);
    Notch_beta2_out = Notch_beta12wn(2);
    Notch_wn_out = Notch_beta12wn(3);
    Notch2_beta1_out = Notch2_beta12wn(1);
    Notch2_beta2_out = Notch2_beta12wn(2);
    Notch2_wn_out = Notch2_beta12wn(3);
    LowPassCutOffFreq_out = LowPassCutOffFreq;
end

== matlab function FAST_11TO14mpers/Controller/Pitch Control/Notch filter/MATLAB Function ==
  data: u input; beta1 input; beta2 input; wn input; y output; Ts input
function y = NotchFilter(u, beta1, beta2, wn, Ts)

persistent u_prev1 u_prev2 y_prev1 y_prev2
if isempty(u_prev1)
    u_prev1 = u;
    u_prev2 = u;
    y_prev1 = u;
    y_prev2 = u;
end

if any([beta1 beta2 wn] == 0)
    y = u;
else
    % Prepare filter elements from current input
    K = 2/Ts;
    Part1 = (K^2 + 2*wn*beta1 * K + wn^2) / (K^2 + 2*wn*beta2 * K + wn^2);
    Part2 = (2 * wn^2 - 2 * K^2)  / (K^2 + 2*wn*beta2 * K + wn^2);
    Part3 = (K^2 - 2*wn*beta1 * K + wn^2) / (K^2 + 2*wn*beta2 * K + wn^2);
    Part4 = (2 * wn^2 - 2 * K^2)  / (K^2 + 2*wn*beta2 * K + wn^2);
    Part5 = (K^2 - 2*wn*beta2* K + wn^2)/ (K^2 + 2*wn*beta2 * K + wn^2);
    
    % Compute filter output
    y = Part1*u + Part2*u_prev1 + Part3*u_prev2 - Part4*y_prev1 - Part5*y_prev2;
    
    % Save signals for next time step
    u_prev2 = u_prev1;
    u_prev1 = u;
    
    y_prev2 = y_prev1;
    y_prev1 = y;
end

== matlab function FAST_11TO14mpers/Controller/Pitch Control/Low-pass filter/Second-order low-pass filter ==
  data: u input; wn input; Damp input; y output; Ts input
function y = SecLPF(u, wn, Damp, Ts)

persistent y_prev1 y_prev2 u_prev1 u_prev2

if isempty(u_prev1)
    y_prev1 = u;
    y_prev2 = u;
    u_prev1 = u;
    u_prev2 = u;
end

y = 1/(4+4*Ts*Damp*wn+Ts^2*wn^2) * ( (8-2*Ts^2*wn^2)*y_prev1 + ...
    (-4+4*Ts*Damp*wn-Ts^2*wn^2)*y_prev2 + (Ts^2*wn^2)*u ...
    + (2*Ts^2*wn^2)*u_prev1 + (Ts^2*wn^2)*u_prev2 );

u_prev2   = u_prev1;
u_prev1   = u;
y_prev2  = y_prev1;
y_prev1  = y;

== matlab function FAST_11TO14mpers/Controller/Pitch Control/Low-pass filter/First-order low-pass filter ==
  data: u input; wn input; y output; Ts input
function y = FirstLPF(u, wn, Ts)

persistent y_prev1 u_prev1

if isempty(u_prev1)
    y_prev1 = u;
    u_prev1 = u;
end

y = (Ts*wn*u + Ts*wn*u_prev1 - (Ts*wn-2.0)*y_prev1)/(Ts*wn+2.0);

u_prev1   = u;
y_prev1  = y;

== matlab function FAST_11TO14mpers/Controller/Torque Control/Low-pass filter/First-order low-pass filter ==
  data: u input; wn input; y output; Ts input
function y = FirstLPF(u, wn, Ts)

persistent y_prev1 u_prev1

if isempty(u_prev1)
    y_prev1 = u;
    u_prev1 = u;
end

y = (Ts*wn*u + Ts*wn*u_prev1 - (Ts*wn-2.0)*y_prev1)/(Ts*wn+2.0);

u_prev1   = u;
y_prev1  = y;

== matlab function FAST_11TO14mpers/Controller/Pitch Control/Notch filter1/MATLAB Function ==
  data: u input; beta1 input; beta2 input; wn input; y output; Ts input
function y = NotchFilter(u, beta1, beta2, wn, Ts)

persistent u_prev1 u_prev2 y_prev1 y_prev2
if isempty(u_prev1)
    u_prev1 = u;
    u_prev2 = u;
    y_prev1 = u;
    y_prev2 = u;
end

if any([beta1 beta2 wn] == 0)
    y = u;
else
    % Prepare filter elements from current input
    K = 2/Ts;
    Part1 = (K^2 + 2*wn*beta1 * K + wn^2) / (K^2 + 2*wn*beta2 * K + wn^2);
    Part2 = (2 * wn^2 - 2 * K^2)  / (K^2 + 2*wn*beta2 * K + wn^2);
    Part3 = (K^2 - 2*wn*beta1 * K + wn^2) / (K^2 + 2*wn*beta2 * K + wn^2);
    Part4 = (2 * wn^2 - 2 * K^2)  / (K^2 + 2*wn*beta2 * K + wn^2);
    Part5 = (K^2 - 2*wn*beta2* K + wn^2)/ (K^2 + 2*wn*beta2 * K + wn^2);
    
    % Compute filter output
    y = Part1*u + Part2*u_prev1 + Part3*u_prev2 - Part4*y_prev1 - Part5*y_prev2;
    
    % Save signals for next time step
    u_prev2 = u_prev1;
    u_prev1 = u;
    
    y_prev2 = y_prev1;
    y_prev1 = y;
end
